simulink model "ferrucci299571_assign1_complete"  (R2026a)
settings: Solver=ode14x  StopTime=simTime  FixedStep=fixedStepSize
undefined symbols (not defined in the file or in its folder): RW
libraries: fl_lib x36, nesl_utility x12, ee_lib x3
settings Model: Creator=ferru  LastModifiedBy=ferru

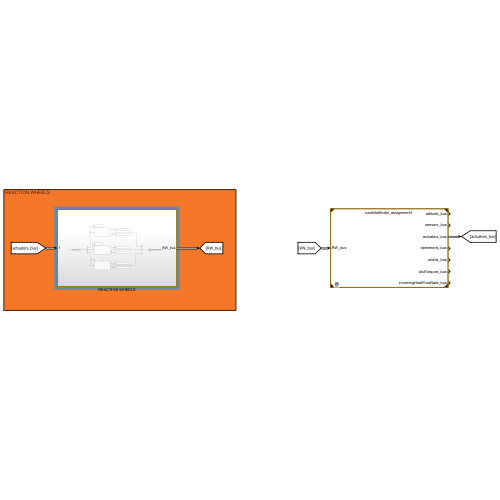
[thumbnail: Simulink's stored preview of the top-level diagram]
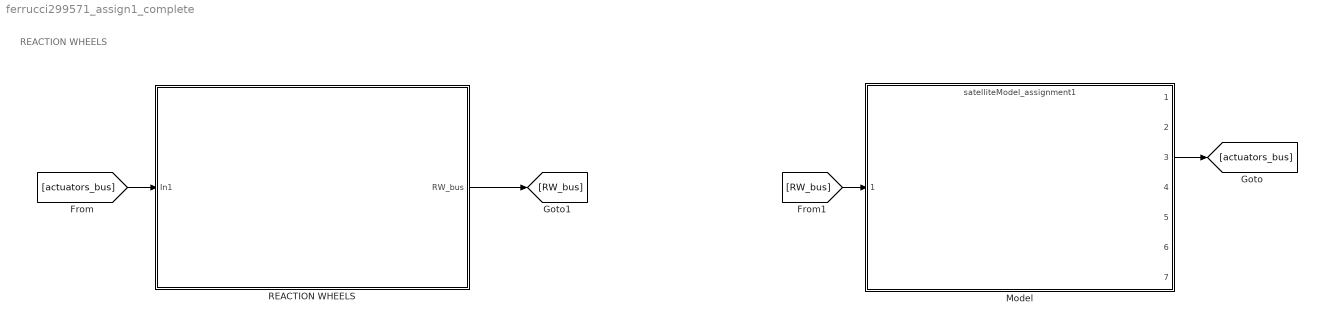
== system ferrucci299571_assign1_complete ==
  note: REACTION WHEELS
  Model : ModelReference  ModelNameDialog=satelliteModel_assignment1.slxp  ModelReferenceVersion=4.59  CopyOfModelProtected=on
  REACTION WHEELS : Subsystem
  wires:
  Model/3 -> [actuators_bus]
  [RW_bus] -> Model/1
  [actuators_bus] -> REACTION WHEELS/1(In1)
  REACTION WHEELS/1(RW_bus) -> [RW_bus]

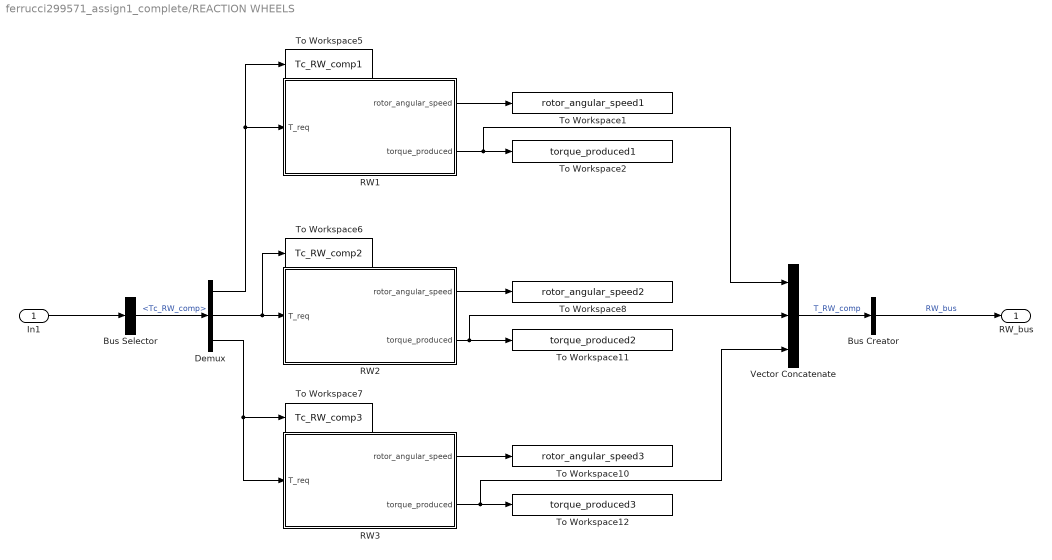
== system ferrucci299571_assign1_complete/REACTION WHEELS ==
  In1 : Inport
  Bus Creator : BusCreator  Inputs=1
  Bus Selector : BusSelector  OutputSignals=RW_bus.Tc_RW_comp
  Demux : Demux  Outputs=3
  RW1 : Subsystem
  RW2 : Subsystem
  RW3 : Subsystem
  To Workspace1 : ToWorkspace  VariableName=rotor_angular_speed1  SampleTime=-1
      settings: Save2DSignal=2-D array (concatenate along first dimension)
  To Workspace10 : ToWorkspace  VariableName=rotor_angular_speed3  SampleTime=-1
      settings: Save2DSignal=2-D array (concatenate along first dimension)
  To Workspace11 : ToWorkspace  VariableName=torque_produced2  SampleTime=-1
      settings: Save2DSignal=2-D array (concatenate along first dimension)
  To Workspace12 : ToWorkspace  VariableName=torque_produced3  SampleTime=-1
      settings: Save2DSignal=2-D array (concatenate along first dimension)
  To Workspace2 : ToWorkspace  VariableName=torque_produced1  SampleTime=-1
      settings: Save2DSignal=2-D array (concatenate along first dimension)
  To Workspace5 : ToWorkspace  VariableName=Tc_RW_comp1  SampleTime=-1
      settings: Save2DSignal=2-D array (concatenate along first dimension)
  To Workspace6 : ToWorkspace  VariableName=Tc_RW_comp2  SampleTime=-1
      settings: Save2DSignal=2-D array (concatenate along first dimension)
  To Workspace7 : ToWorkspace  VariableName=Tc_RW_comp3  SampleTime=-1
      settings: Save2DSignal=2-D array (concatenate along first dimension)
  To Workspace8 : ToWorkspace  VariableName=rotor_angular_speed2  SampleTime=-1
      settings: Save2DSignal=2-D array (concatenate along first dimension)
  Vector Concatenate : Concatenate  NumInputs=3  Mode=Multidimensional array
  RW_bus : Outport
  wires:
  Vector Concatenate/1 -> Bus Creator/1  "T_RW_comp"
  Demux/1 -> To Workspace5/1, RW1/1(T_req)
  Demux/3 -> RW3/1(T_req), To Workspace7/1
  Bus Creator/1 -> RW_bus/1  "RW_bus"
  RW3/2(torque_produced) -> Vector Concatenate/3, To Workspace12/1
  Bus Selector/1 -> Demux/1  "<Tc_RW_comp>"
  RW1/1(rotor_angular_speed) -> To Workspace1/1
  RW3/1(rotor_angular_speed) -> To Workspace10/1
  Demux/2 -> RW2/1(T_req), To Workspace6/1
  RW2/2(torque_produced) -> Vector Concatenate/2, To Workspace11/1
  RW2/1(rotor_angular_speed) -> To Workspace8/1
  RW1/2(torque_produced) -> Vector Concatenate/1, To Workspace2/1
  In1/1 -> Bus Selector/1

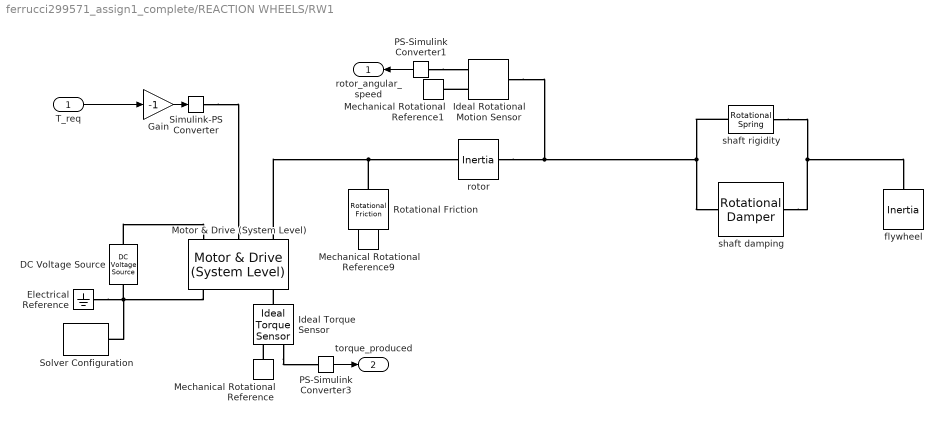
== system ferrucci299571_assign1_complete/REACTION WHEELS/RW1 ==
  T_req : Inport
  DC Voltage Source : fl_lib/Electrical/Electrical Sources/DC Voltage Source  v0=10 V
  Electrical Reference : fl_lib/Electrical/Electrical Elements/Electrical Reference
  Gain : Gain  Gain=-1
  Ideal Rotational Motion Sensor : fl_lib/Mechanical/Mechanical Sensors/Ideal Rotational Motion Sensor  reference=foundation.enum.MeasurementReference.difference  acceleration_port=false  velocity_port=true  position_port=false  wrap_angle=false  offset=0 rad
  Ideal Torque Sensor : fl_lib/Mechanical/Mechanical Sensors/Ideal Torque Sensor
  Mechanical Rotational Reference : fl_lib/Mechanical/Rotational Elements/Mechanical Rotational Reference
  Mechanical Rotational Reference1 : fl_lib/Mechanical/Rotational Elements/Mechanical Rotational Reference
  Mechanical Rotational Reference9 : fl_lib/Mechanical/Rotational Elements/Mechanical Rotational Reference
  Motor & Drive (System Level) : ee_lib/Electromechanical/Motor & Drive (System Level)  torque_speed_param=ee.enum.electromech.envelope.tabulated  overtorque_param=ee.enum.electromech.overtorque.no  T_t=RW.torque_envelope_val mN*m  T_t_intermittent=[.36, .32, .28, 0] N*m  T_t_2D=[.09, .09, .09; .08, .08, .08; .07, .07, .07; 0, 0, 0] N*m  T_t_intermittent_2D=[.36, .36, .36; .32, .32, .32; .28, .28, .28; 0, 0, 0] N*m  w_t=RW.torque_envelope_omega rad/s  vdc_t=[6, 12, 24] V  torque_max=0.1 N*m  power_max=30 W  torque_max_intermittent=0.4 N*m  power_max_intermittent=120 W  time_overtorque=30 s  time_recover=60 s  Tc=RW.torque_control_tc s  EnableSwitch=false  losses_param=ee.enum.electromech.motorAndDrive.lossParameterization.TabulatedEfficiencyDataAsAFunctionOfSpeedAndTorque  eff=100  w_eff=3750 rpm  T_eff=0.08 N*m  Piron=0 W  Pbase=0 W  w_eff_vec=RW.efficiency_omega rad/s  T_eff_vec=RW.efficiency_torque mN*m  v_eff_vec=[100, 250, 400] V  losses_mat=[1.49, 1.67, 2.21, 3.1; .42, .69, 1.14, 2.03; .06, .24, .78, 1.68; .42, .69, 1.14, 2.03; 1.49, 1.67, 2.21, 3.1] W  efficiency_mat=RW.efficiency_mat  losses_mat_3D=ones(5, 4, 3) W  efficiency_mat_3D=95 * ones(5, 4, 3)  Res=0 Ohm  J=RW.rotor_inertia_motor kg*m^2  lam=RW.rotor_damping N*m*s/rad  speed0=0 rpm  faulted_specify=off  faulted_priority=None  faulted=0  faulted_nominal_specify=off  faulted_nominal_value=1  faulted_nominal_unit=1  isSwitchedOff_specify=off  isSwitchedOff_priority=None  isSwitchedOff=0  isSwitchedOff_nominal_specify=off  isSwitchedOff_nominal_value=1  isSwitchedOff_nominal_unit=1  torqueLimitContinuous_specify=off  torqueLimitContinuous_priority=None  torqueLimitContinuous=0 N*m  torqueLimitContinuous_nominal_specify=off  torqueLimitContinuous_nominal_value=1  torqueLimitContinuous_nominal_unit=N*m  TabulateLossesForMultipleTemperatures=false  alpha=3.93e-3 1/K  Tmeas=25 degC  TmeasVec=[25, 75, 125] degC  Tmeas2=125 degC  losses_mat_T2=[1.49, 1.74, 2.49, 3.74; .42, .67, 1.42, 2.67; .06, .31, 1.06, 2.31; .42, .67, 1.42, 2.67; 1.49, 1.74, 2.49, 3.74] W  efficiency_mat_T2=[95, 95, 95, 95; 95, 95, 95, 95; 95, 95, 95, 95; 95, 95, 95, 95; 95, 95, 95, 95]  losses_mat_3D_T2=ones(5, 4, 3) W  efficiency_mat_3D_T2=95 * ones(5, 4, 3)  lossesMatMultipleTemperatures=ones(5, 4, 3) W  efficiencyMatMultipleTemperatures=95 * ones(5, 4, 3)  lossesMat4DMultipleTemperatures=ones(5, 4, 3, 3) W  efficiencyMat4DMultipleTemperatures=95 * ones(5, 4, 3, 3)  thermal_mass=100 J/K  initial_temperature=25 degC
  PS-Simulink Converter1 : nesl_utility/PS-Simulink Converter  PhysicalDomain=network_engine_domain  SubClassName=ps_output  LeftPortType=input  RightPortType=output  PseudoPeriodic=off  Frequencies=[]  VectorFormat=inherit  Unit=rad/s  AffineConversion=off
  PS-Simulink Converter3 : nesl_utility/PS-Simulink Converter  PhysicalDomain=network_engine_domain  SubClassName=ps_output  LeftPortType=input  RightPortType=output  PseudoPeriodic=off  Frequencies=[]  VectorFormat=inherit  Unit=N*m  AffineConversion=off
  Rotational Friction : fl_lib/Mechanical/Rotational Elements/Rotational Friction  brkwy_trq=RW.breakaway_friction_torque N*m  brkwy_vel=RW.breakaway_friction_velocity rad/s  Col_trq=RW.coulomb_friction_torque N*m  visc_coef=RW.viscous_friction_coeff N*m*s/rad  w_specify=off  w_priority=None  w=0 rad/s  w_nominal_specify=off  w_nominal_value=1  w_nominal_unit=rad/s  t_specify=off  t_priority=None  t=0 N*m  t_nominal_specify=off  t_nominal_value=1  t_nominal_unit=N*m
  Simulink-PS Converter : nesl_utility/Simulink-PS Converter  PhysicalDomain=network_engine_domain  SubClassName=ps_input  LeftPortType=input  RightPortType=output  PseudoPeriodic=off  Frequencies=[]  NoiseDistribution=none  NoiseParameters=[]  Unit=N*m  AffineConversion=off  FilteringAndDerivatives=provide  SimscapeFilterOrder=1  InputFilterTimeConstant=0.001  UdotUserProvided=0
  Solver Configuration : nesl_utility/Solver Configuration  PhysicalDomain=network_engine_domain  SubClassName=solver  LeftPortType=input  RightPortType=generic  Tones=[]  Harmonics=[]  SimulateNoise=off  Profile=off  UseLocalSampling=off  EnableSwitchedLinearOptims=on  FrequencyDomain=off  UseCCode=off  RelTol=0.001  AbsTol=0.001  MinStep=1e-09  ToWorkspace=off  RevertToSquareIcSolve=off  NumHomotopyIterations=100  PhasorMode=off  PhasorModeNumHarmonics=1  ConsistencySolver=NEWTON_XTOL_AFTER_FTOL  CanonicalOrdering=CANONICAL  OptimizeIntermediates=OPTIMIZED  IndexReductionMethod=DerivativeReplacement  DoDC=off  ResidualTolerance=1e-09  ConsistencyTolSource=GLOBAL  ConsistencyAbsTol=0.001  ConsistencyRelTol=0.001  ConsistencyTolFactor=0.001  UseLocalSolver=off  LocalSolverChoice=NE_BACKWARD_EULER_ADVANCER  ResolveIndetEquations=on  FunctionEvalNumThread=1  LocalSolverSampleTime=0.001  DoFixedCost=off  MaxNonlinIter=3  MaxModeIter=2  ComputeImpulses=off  ImpulseIterations=2  LinearAlgebra=auto  LinearAlgebraNumThread=0  EquationFormulation=NE_TIME_EF  DelaysMemoryBudget=1024  AutomaticFiltering=on  FilteringTimeConstant=0.001  PartitionStorageMethod=AS_NEEDED  PartitionMemoryBudget=1024  PartitionMethod=ROBUST  MultibodyUseLocalSolver=off  MultibodyLocalSolverChoice=ODE1  MultibodyLocalSolverSampleTime=0.001
  flywheel : fl_lib/Mechanical/Rotational Elements/Inertia  inertia=RW.flywheel_inertia kg*m^2  num_ports=foundation.enum.numPorts2.one  w_specify=off  w_priority=High  w=0 rad/s  w_nominal_specify=off  w_nominal_value=1  w_nominal_unit=rad/s  t_specify=off  t_priority=None  t=0 N*m  t_nominal_specify=off  t_nominal_value=1  t_nominal_unit=N*m
  rotor : fl_lib/Mechanical/Rotational Elements/Inertia  inertia=RW.rotor_inertia kg*m^2  num_ports=foundation.enum.numPorts2.two  w_specify=off  w_priority=High  w=0 rad/s  w_nominal_specify=off  w_nominal_value=1  w_nominal_unit=rad/s  t_specify=off  t_priority=None  t=0 N*m  t_nominal_specify=off  t_nominal_value=1  t_nominal_unit=N*m
  shaft damping : fl_lib/Mechanical/Rotational Elements/Rotational Damper  D=RW.shaft_damping_coeff N*m*s/rad  w_specify=off  w_priority=None  w=0 rad/s  w_nominal_specify=off  w_nominal_value=1  w_nominal_unit=rad/s  t_specify=off  t_priority=None  t=0 N*m  t_nominal_specify=off  t_nominal_value=1  t_nominal_unit=N*m
  shaft rigidity : fl_lib/Mechanical/Rotational Elements/Rotational Spring  spr_rate=RW.shaft_spring_rate N*m/rad  w_specify=off  w_priority=None  w=0 rad/s  w_nominal_specify=off  w_nominal_value=1  w_nominal_unit=rad/s  t_specify=off  t_priority=None  t=0 N*m  t_nominal_specify=off  t_nominal_value=1  t_nominal_unit=N*m  phi_specify=off  phi_priority=High  phi=0 rad  phi_nominal_specify=off  phi_nominal_value=1  phi_nominal_unit=rad
  rotor_angular_speed : Outport
  torque_produced : Outport  Port=2
  wires:
  Gain/1 -> Simulink-PS Converter/1
  PS-Simulink Converter3/1 -> torque_produced/1
  PS-Simulink Converter1/1 -> rotor_angular_speed/1
  T_req/1 -> Gain/1
  connections:
  DC Voltage Source/RConn1 -- Electrical Reference/LConn1 -- Motor & Drive (System Level)/RConn1 -- Solver Configuration/RConn1
  Mechanical Rotational Reference9/LConn1 -- Rotational Friction/RConn1
  Ideal Torque Sensor/RConn2 -- PS-Simulink Converter3/LConn1
  shaft rigidity/LConn1 -- flywheel/LConn1 -- shaft damping/LConn1
  Rotational Friction/LConn1 -- Motor & Drive (System Level)/LConn3 -- rotor/RConn1
  Simulink-PS Converter/RConn1 -- Motor & Drive (System Level)/LConn2
  PS-Simulink Converter1/LConn1 -- Ideal Rotational Motion Sensor/RConn2
  Mechanical Rotational Reference/LConn1 -- Ideal Torque Sensor/RConn1
  Ideal Rotational Motion Sensor/RConn1 -- Mechanical Rotational Reference1/LConn1
  DC Voltage Source/LConn1 -- Motor & Drive (System Level)/LConn1
  rotor/LConn1 -- Ideal Rotational Motion Sensor/LConn1 -- shaft rigidity/RConn1 -- shaft damping/RConn1
  Ideal Torque Sensor/LConn1 -- Motor & Drive (System Level)/RConn3

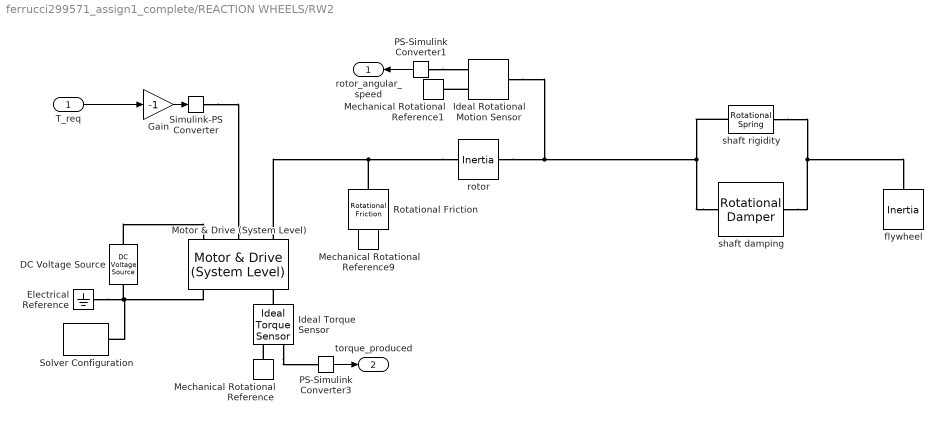
== system ferrucci299571_assign1_complete/REACTION WHEELS/RW2 ==
  T_req : Inport
  DC Voltage Source : fl_lib/Electrical/Electrical Sources/DC Voltage Source  v0=10 V
  Electrical Reference : fl_lib/Electrical/Electrical Elements/Electrical Reference
  Gain : Gain  Gain=-1
  Ideal Rotational Motion Sensor : fl_lib/Mechanical/Mechanical Sensors/Ideal Rotational Motion Sensor  reference=foundation.enum.MeasurementReference.difference  acceleration_port=false  velocity_port=true  position_port=false  wrap_angle=false  offset=0 rad
  Ideal Torque Sensor : fl_lib/Mechanical/Mechanical Sensors/Ideal Torque Sensor
  Mechanical Rotational Reference : fl_lib/Mechanical/Rotational Elements/Mechanical Rotational Reference
  Mechanical Rotational Reference1 : fl_lib/Mechanical/Rotational Elements/Mechanical Rotational Reference
  Mechanical Rotational Reference9 : fl_lib/Mechanical/Rotational Elements/Mechanical Rotational Reference
  Motor & Drive (System Level) : ee_lib/Electromechanical/Motor & Drive (System Level)  torque_speed_param=ee.enum.electromech.envelope.tabulated  overtorque_param=ee.enum.electromech.overtorque.no  T_t=RW.torque_envelope_val mN*m  T_t_intermittent=[.36, .32, .28, 0] N*m  T_t_2D=[.09, .09, .09; .08, .08, .08; .07, .07, .07; 0, 0, 0] N*m  T_t_intermittent_2D=[.36, .36, .36; .32, .32, .32; .28, .28, .28; 0, 0, 0] N*m  w_t=RW.torque_envelope_omega rad/s  vdc_t=[6, 12, 24] V  torque_max=0.1 N*m  power_max=30 W  torque_max_intermittent=0.4 N*m  power_max_intermittent=120 W  time_overtorque=30 s  time_recover=60 s  Tc=RW.torque_control_tc s  EnableSwitch=false  losses_param=ee.enum.electromech.motorAndDrive.lossParameterization.TabulatedEfficiencyDataAsAFunctionOfSpeedAndTorque  eff=100  w_eff=3750 rpm  T_eff=0.08 N*m  Piron=0 W  Pbase=0 W  w_eff_vec=RW.efficiency_omega rad/s  T_eff_vec=RW.efficiency_torque mN*m  v_eff_vec=[100, 250, 400] V  losses_mat=[1.49, 1.67, 2.21, 3.1; .42, .69, 1.14, 2.03; .06, .24, .78, 1.68; .42, .69, 1.14, 2.03; 1.49, 1.67, 2.21, 3.1] W  efficiency_mat=RW.efficiency_mat  losses_mat_3D=ones(5, 4, 3) W  efficiency_mat_3D=95 * ones(5, 4, 3)  Res=0 Ohm  J=RW.rotor_inertia_motor kg*m^2  lam=RW.rotor_damping N*m*s/rad  speed0=0 rpm  faulted_specify=off  faulted_priority=None  faulted=0  faulted_nominal_specify=off  faulted_nominal_value=1  faulted_nominal_unit=1  isSwitchedOff_specify=off  isSwitchedOff_priority=None  isSwitchedOff=0  isSwitchedOff_nominal_specify=off  isSwitchedOff_nominal_value=1  isSwitchedOff_nominal_unit=1  torqueLimitContinuous_specify=off  torqueLimitContinuous_priority=None  torqueLimitContinuous=0 N*m  torqueLimitContinuous_nominal_specify=off  torqueLimitContinuous_nominal_value=1  torqueLimitContinuous_nominal_unit=N*m  TabulateLossesForMultipleTemperatures=false  alpha=3.93e-3 1/K  Tmeas=25 degC  TmeasVec=[25, 75, 125] degC  Tmeas2=125 degC  losses_mat_T2=[1.49, 1.74, 2.49, 3.74; .42, .67, 1.42, 2.67; .06, .31, 1.06, 2.31; .42, .67, 1.42, 2.67; 1.49, 1.74, 2.49, 3.74] W  efficiency_mat_T2=[95, 95, 95, 95; 95, 95, 95, 95; 95, 95, 95, 95; 95, 95, 95, 95; 95, 95, 95, 95]  losses_mat_3D_T2=ones(5, 4, 3) W  efficiency_mat_3D_T2=95 * ones(5, 4, 3)  lossesMatMultipleTemperatures=ones(5, 4, 3) W  efficiencyMatMultipleTemperatures=95 * ones(5, 4, 3)  lossesMat4DMultipleTemperatures=ones(5, 4, 3, 3) W  efficiencyMat4DMultipleTemperatures=95 * ones(5, 4, 3, 3)  thermal_mass=100 J/K  initial_temperature=25 degC
  PS-Simulink Converter1 : nesl_utility/PS-Simulink Converter  PhysicalDomain=network_engine_domain  SubClassName=ps_output  LeftPortType=input  RightPortType=output  PseudoPeriodic=off  Frequencies=[]  VectorFormat=inherit  Unit=rad/s  AffineConversion=off
  PS-Simulink Converter3 : nesl_utility/PS-Simulink Converter  PhysicalDomain=network_engine_domain  SubClassName=ps_output  LeftPortType=input  RightPortType=output  PseudoPeriodic=off  Frequencies=[]  VectorFormat=inherit  Unit=N*m  AffineConversion=off
  Rotational Friction : fl_lib/Mechanical/Rotational Elements/Rotational Friction  brkwy_trq=RW.breakaway_friction_torque N*m  brkwy_vel=RW.breakaway_friction_velocity rad/s  Col_trq=RW.coulomb_friction_torque N*m  visc_coef=RW.viscous_friction_coeff N*m*s/rad  w_specify=off  w_priority=None  w=0 rad/s  w_nominal_specify=off  w_nominal_value=1  w_nominal_unit=rad/s  t_specify=off  t_priority=None  t=0 N*m  t_nominal_specify=off  t_nominal_value=1  t_nominal_unit=N*m
  Simulink-PS Converter : nesl_utility/Simulink-PS Converter  PhysicalDomain=network_engine_domain  SubClassName=ps_input  LeftPortType=input  RightPortType=output  PseudoPeriodic=off  Frequencies=[]  NoiseDistribution=none  NoiseParameters=[]  Unit=N*m  AffineConversion=off  FilteringAndDerivatives=provide  SimscapeFilterOrder=1  InputFilterTimeConstant=0.001  UdotUserProvided=0
  Solver Configuration : nesl_utility/Solver Configuration  PhysicalDomain=network_engine_domain  SubClassName=solver  LeftPortType=input  RightPortType=generic  Tones=[]  Harmonics=[]  SimulateNoise=off  Profile=off  UseLocalSampling=off  EnableSwitchedLinearOptims=on  FrequencyDomain=off  UseCCode=off  RelTol=0.001  AbsTol=0.001  MinStep=1e-09  ToWorkspace=off  RevertToSquareIcSolve=off  NumHomotopyIterations=100  PhasorMode=off  PhasorModeNumHarmonics=1  ConsistencySolver=NEWTON_XTOL_AFTER_FTOL  CanonicalOrdering=CANONICAL  OptimizeIntermediates=OPTIMIZED  IndexReductionMethod=DerivativeReplacement  DoDC=off  ResidualTolerance=1e-09  ConsistencyTolSource=GLOBAL  ConsistencyAbsTol=0.001  ConsistencyRelTol=0.001  ConsistencyTolFactor=0.001  UseLocalSolver=off  LocalSolverChoice=NE_BACKWARD_EULER_ADVANCER  ResolveIndetEquations=on  FunctionEvalNumThread=1  LocalSolverSampleTime=0.001  DoFixedCost=off  MaxNonlinIter=3  MaxModeIter=2  ComputeImpulses=off  ImpulseIterations=2  LinearAlgebra=auto  LinearAlgebraNumThread=0  EquationFormulation=NE_TIME_EF  DelaysMemoryBudget=1024  AutomaticFiltering=on  FilteringTimeConstant=0.001  PartitionStorageMethod=AS_NEEDED  PartitionMemoryBudget=1024  PartitionMethod=ROBUST  MultibodyUseLocalSolver=off  MultibodyLocalSolverChoice=ODE1  MultibodyLocalSolverSampleTime=0.001
  flywheel : fl_lib/Mechanical/Rotational Elements/Inertia  inertia=RW.flywheel_inertia kg*m^2  num_ports=foundation.enum.numPorts2.one  w_specify=off  w_priority=High  w=0 rad/s  w_nominal_specify=off  w_nominal_value=1  w_nominal_unit=rad/s  t_specify=off  t_priority=None  t=0 N*m  t_nominal_specify=off  t_nominal_value=1  t_nominal_unit=N*m
  rotor : fl_lib/Mechanical/Rotational Elements/Inertia  inertia=RW.rotor_inertia kg*m^2  num_ports=foundation.enum.numPorts2.two  w_specify=off  w_priority=High  w=0 rad/s  w_nominal_specify=off  w_nominal_value=1  w_nominal_unit=rad/s  t_specify=off  t_priority=None  t=0 N*m  t_nominal_specify=off  t_nominal_value=1  t_nominal_unit=N*m
  shaft damping : fl_lib/Mechanical/Rotational Elements/Rotational Damper  D=RW.shaft_damping_coeff N*m*s/rad  w_specify=off  w_priority=None  w=0 rad/s  w_nominal_specify=off  w_nominal_value=1  w_nominal_unit=rad/s  t_specify=off  t_priority=None  t=0 N*m  t_nominal_specify=off  t_nominal_value=1  t_nominal_unit=N*m
  shaft rigidity : fl_lib/Mechanical/Rotational Elements/Rotational Spring  spr_rate=RW.shaft_spring_rate N*m/rad  w_specify=off  w_priority=None  w=0 rad/s  w_nominal_specify=off  w_nominal_value=1  w_nominal_unit=rad/s  t_specify=off  t_priority=None  t=0 N*m  t_nominal_specify=off  t_nominal_value=1  t_nominal_unit=N*m  phi_specify=off  phi_priority=High  phi=0 rad  phi_nominal_specify=off  phi_nominal_value=1  phi_nominal_unit=rad
  rotor_angular_speed : Outport
  torque_produced : Outport  Port=2
  wires:
  T_req/1 -> Gain/1
  PS-Simulink Converter1/1 -> rotor_angular_speed/1
  PS-Simulink Converter3/1 -> torque_produced/1
  Gain/1 -> Simulink-PS Converter/1
  connections:
  Ideal Torque Sensor/LConn1 -- Motor & Drive (System Level)/RConn3
  shaft damping/RConn1 -- shaft rigidity/RConn1 -- Ideal Rotational Motion Sensor/LConn1 -- rotor/LConn1
  DC Voltage Source/LConn1 -- Motor & Drive (System Level)/LConn1
  Ideal Rotational Motion Sensor/RConn1 -- Mechanical Rotational Reference1/LConn1
  Mechanical Rotational Reference/LConn1 -- Ideal Torque Sensor/RConn1
  PS-Simulink Converter1/LConn1 -- Ideal Rotational Motion Sensor/RConn2
  Simulink-PS Converter/RConn1 -- Motor & Drive (System Level)/LConn2
  rotor/RConn1 -- Motor & Drive (System Level)/LConn3 -- Rotational Friction/LConn1
  shaft damping/LConn1 -- flywheel/LConn1 -- shaft rigidity/LConn1
  Ideal Torque Sensor/RConn2 -- PS-Simulink Converter3/LConn1
  Mechanical Rotational Reference9/LConn1 -- Rotational Friction/RConn1
  Solver Configuration/RConn1 -- Motor & Drive (System Level)/RConn1 -- Electrical Reference/LConn1 -- DC Voltage Source/RConn1

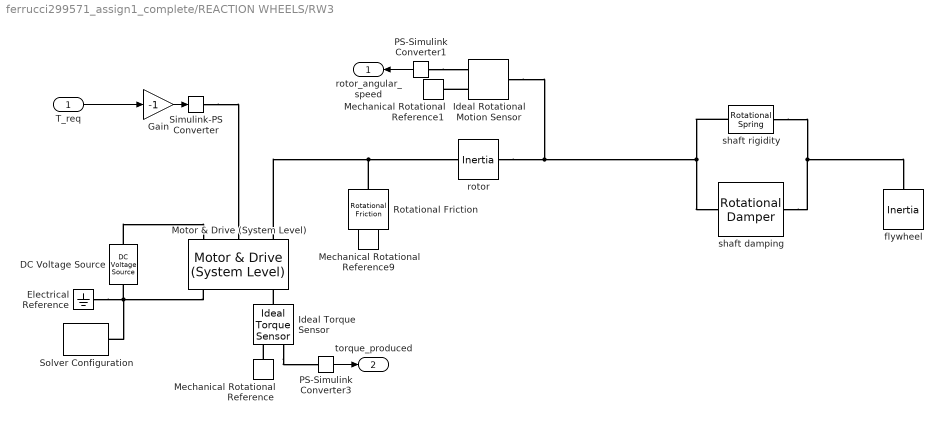
== system ferrucci299571_assign1_complete/REACTION WHEELS/RW3 ==
  T_req : Inport
  DC Voltage Source : fl_lib/Electrical/Electrical Sources/DC Voltage Source  v0=10 V
  Electrical Reference : fl_lib/Electrical/Electrical Elements/Electrical Reference
  Gain : Gain  Gain=-1
  Ideal Rotational Motion Sensor : fl_lib/Mechanical/Mechanical Sensors/Ideal Rotational Motion Sensor  reference=foundation.enum.MeasurementReference.difference  acceleration_port=false  velocity_port=true  position_port=false  wrap_angle=false  offset=0 rad
  Ideal Torque Sensor : fl_lib/Mechanical/Mechanical Sensors/Ideal Torque Sensor
  Mechanical Rotational Reference : fl_lib/Mechanical/Rotational Elements/Mechanical Rotational Reference
  Mechanical Rotational Reference1 : fl_lib/Mechanical/Rotational Elements/Mechanical Rotational Reference
  Mechanical Rotational Reference9 : fl_lib/Mechanical/Rotational Elements/Mechanical Rotational Reference
  Motor & Drive (System Level) : ee_lib/Electromechanical/Motor & Drive (System Level)  torque_speed_param=ee.enum.electromech.envelope.tabulated  overtorque_param=ee.enum.electromech.overtorque.no  T_t=RW.torque_envelope_val mN*m  T_t_intermittent=[.36, .32, .28, 0] N*m  T_t_2D=[.09, .09, .09; .08, .08, .08; .07, .07, .07; 0, 0, 0] N*m  T_t_intermittent_2D=[.36, .36, .36; .32, .32, .32; .28, .28, .28; 0, 0, 0] N*m  w_t=RW.torque_envelope_omega rad/s  vdc_t=[6, 12, 24] V  torque_max=0.1 N*m  power_max=30 W  torque_max_intermittent=0.4 N*m  power_max_intermittent=120 W  time_overtorque=30 s  time_recover=60 s  Tc=RW.torque_control_tc s  EnableSwitch=false  losses_param=ee.enum.electromech.motorAndDrive.lossParameterization.TabulatedEfficiencyDataAsAFunctionOfSpeedAndTorque  eff=100  w_eff=3750 rpm  T_eff=0.08 N*m  Piron=0 W  Pbase=0 W  w_eff_vec=RW.efficiency_omega rad/s  T_eff_vec=RW.efficiency_torque mN*m  v_eff_vec=[100, 250, 400] V  losses_mat=[1.49, 1.67, 2.21, 3.1; .42, .69, 1.14, 2.03; .06, .24, .78, 1.68; .42, .69, 1.14, 2.03; 1.49, 1.67, 2.21, 3.1] W  efficiency_mat=RW.efficiency_mat  losses_mat_3D=ones(5, 4, 3) W  efficiency_mat_3D=95 * ones(5, 4, 3)  Res=0 Ohm  J=RW.rotor_inertia_motor kg*m^2  lam=RW.rotor_damping N*m*s/rad  speed0=0 rpm  faulted_specify=off  faulted_priority=None  faulted=0  faulted_nominal_specify=off  faulted_nominal_value=1  faulted_nominal_unit=1  isSwitchedOff_specify=off  isSwitchedOff_priority=None  isSwitchedOff=0  isSwitchedOff_nominal_specify=off  isSwitchedOff_nominal_value=1  isSwitchedOff_nominal_unit=1  torqueLimitContinuous_specify=off  torqueLimitContinuous_priority=None  torqueLimitContinuous=0 N*m  torqueLimitContinuous_nominal_specify=off  torqueLimitContinuous_nominal_value=1  torqueLimitContinuous_nominal_unit=N*m  TabulateLossesForMultipleTemperatures=false  alpha=3.93e-3 1/K  Tmeas=25 degC  TmeasVec=[25, 75, 125] degC  Tmeas2=125 degC  losses_mat_T2=[1.49, 1.74, 2.49, 3.74; .42, .67, 1.42, 2.67; .06, .31, 1.06, 2.31; .42, .67, 1.42, 2.67; 1.49, 1.74, 2.49, 3.74] W  efficiency_mat_T2=[95, 95, 95, 95; 95, 95, 95, 95; 95, 95, 95, 95; 95, 95, 95, 95; 95, 95, 95, 95]  losses_mat_3D_T2=ones(5, 4, 3) W  efficiency_mat_3D_T2=95 * ones(5, 4, 3)  lossesMatMultipleTemperatures=ones(5, 4, 3) W  efficiencyMatMultipleTemperatures=95 * ones(5, 4, 3)  lossesMat4DMultipleTemperatures=ones(5, 4, 3, 3) W  efficiencyMat4DMultipleTemperatures=95 * ones(5, 4, 3, 3)  thermal_mass=100 J/K  initial_temperature=25 degC
  PS-Simulink Converter1 : nesl_utility/PS-Simulink Converter  PhysicalDomain=network_engine_domain  SubClassName=ps_output  LeftPortType=input  RightPortType=output  PseudoPeriodic=off  Frequencies=[]  VectorFormat=inherit  Unit=rad/s  AffineConversion=off
  PS-Simulink Converter3 : nesl_utility/PS-Simulink Converter  PhysicalDomain=network_engine_domain  SubClassName=ps_output  LeftPortType=input  RightPortType=output  PseudoPeriodic=off  Frequencies=[]  VectorFormat=inherit  Unit=N*m  AffineConversion=off
  Rotational Friction : fl_lib/Mechanical/Rotational Elements/Rotational Friction  brkwy_trq=RW.breakaway_friction_torque N*m  brkwy_vel=RW.breakaway_friction_velocity rad/s  Col_trq=RW.coulomb_friction_torque N*m  visc_coef=RW.viscous_friction_coeff N*m*s/rad  w_specify=off  w_priority=None  w=0 rad/s  w_nominal_specify=off  w_nominal_value=1  w_nominal_unit=rad/s  t_specify=off  t_priority=None  t=0 N*m  t_nominal_specify=off  t_nominal_value=1  t_nominal_unit=N*m
  Simulink-PS Converter : nesl_utility/Simulink-PS Converter  PhysicalDomain=network_engine_domain  SubClassName=ps_input  LeftPortType=input  RightPortType=output  PseudoPeriodic=off  Frequencies=[]  NoiseDistribution=none  NoiseParameters=[]  Unit=N*m  AffineConversion=off  FilteringAndDerivatives=provide  SimscapeFilterOrder=1  InputFilterTimeConstant=0.001  UdotUserProvided=0
  Solver Configuration : nesl_utility/Solver Configuration  PhysicalDomain=network_engine_domain  SubClassName=solver  LeftPortType=input  RightPortType=generic  Tones=[]  Harmonics=[]  SimulateNoise=off  Profile=off  UseLocalSampling=off  EnableSwitchedLinearOptims=on  FrequencyDomain=off  UseCCode=off  RelTol=0.001  AbsTol=0.001  MinStep=1e-09  ToWorkspace=off  RevertToSquareIcSolve=off  NumHomotopyIterations=100  PhasorMode=off  PhasorModeNumHarmonics=1  ConsistencySolver=NEWTON_XTOL_AFTER_FTOL  CanonicalOrdering=CANONICAL  OptimizeIntermediates=OPTIMIZED  IndexReductionMethod=DerivativeReplacement  DoDC=off  ResidualTolerance=1e-09  ConsistencyTolSource=GLOBAL  ConsistencyAbsTol=0.001  ConsistencyRelTol=0.001  ConsistencyTolFactor=0.001  UseLocalSolver=off  LocalSolverChoice=NE_BACKWARD_EULER_ADVANCER  ResolveIndetEquations=on  FunctionEvalNumThread=1  LocalSolverSampleTime=0.001  DoFixedCost=off  MaxNonlinIter=3  MaxModeIter=2  ComputeImpulses=off  ImpulseIterations=2  LinearAlgebra=auto  LinearAlgebraNumThread=0  EquationFormulation=NE_TIME_EF  DelaysMemoryBudget=1024  AutomaticFiltering=on  FilteringTimeConstant=0.001  PartitionStorageMethod=AS_NEEDED  PartitionMemoryBudget=1024  PartitionMethod=ROBUST  MultibodyUseLocalSolver=off  MultibodyLocalSolverChoice=ODE1  MultibodyLocalSolverSampleTime=0.001
  flywheel : fl_lib/Mechanical/Rotational Elements/Inertia  inertia=RW.flywheel_inertia kg*m^2  num_ports=foundation.enum.numPorts2.one  w_specify=off  w_priority=High  w=0 rad/s  w_nominal_specify=off  w_nominal_value=1  w_nominal_unit=rad/s  t_specify=off  t_priority=None  t=0 N*m  t_nominal_specify=off  t_nominal_value=1  t_nominal_unit=N*m
  rotor : fl_lib/Mechanical/Rotational Elements/Inertia  inertia=RW.rotor_inertia kg*m^2  num_ports=foundation.enum.numPorts2.two  w_specify=off  w_priority=High  w=0 rad/s  w_nominal_specify=off  w_nominal_value=1  w_nominal_unit=rad/s  t_specify=off  t_priority=None  t=0 N*m  t_nominal_specify=off  t_nominal_value=1  t_nominal_unit=N*m
  shaft damping : fl_lib/Mechanical/Rotational Elements/Rotational Damper  D=RW.shaft_damping_coeff N*m*s/rad  w_specify=off  w_priority=None  w=0 rad/s  w_nominal_specify=off  w_nominal_value=1  w_nominal_unit=rad/s  t_specify=off  t_priority=None  t=0 N*m  t_nominal_specify=off  t_nominal_value=1  t_nominal_unit=N*m
  shaft rigidity : fl_lib/Mechanical/Rotational Elements/Rotational Spring  spr_rate=RW.shaft_spring_rate N*m/rad  w_specify=off  w_priority=None  w=0 rad/s  w_nominal_specify=off  w_nominal_value=1  w_nominal_unit=rad/s  t_specify=off  t_priority=None  t=0 N*m  t_nominal_specify=off  t_nominal_value=1  t_nominal_unit=N*m  phi_specify=off  phi_priority=High  phi=0 rad  phi_nominal_specify=off  phi_nominal_value=1  phi_nominal_unit=rad
  rotor_angular_speed : Outport
  torque_produced : Outport  Port=2
  wires:
  Gain/1 -> Simulink-PS Converter/1
  PS-Simulink Converter3/1 -> torque_produced/1
  PS-Simulink Converter1/1 -> rotor_angular_speed/1
  T_req/1 -> Gain/1
  connections:
  DC Voltage Source/RConn1 -- Electrical Reference/LConn1 -- Motor & Drive (System Level)/RConn1 -- Solver Configuration/RConn1
  Mechanical Rotational Reference9/LConn1 -- Rotational Friction/RConn1
  Ideal Torque Sensor/RConn2 -- PS-Simulink Converter3/LConn1
  shaft rigidity/LConn1 -- flywheel/LConn1 -- shaft damping/LConn1
  Rotational Friction/LConn1 -- Motor & Drive (System Level)/LConn3 -- rotor/RConn1
  Simulink-PS Converter/RConn1 -- Motor & Drive (System Level)/LConn2
  PS-Simulink Converter1/LConn1 -- Ideal Rotational Motion Sensor/RConn2
  Mechanical Rotational Reference/LConn1 -- Ideal Torque Sensor/RConn1
  Ideal Rotational Motion Sensor/RConn1 -- Mechanical Rotational Reference1/LConn1
  DC Voltage Source/LConn1 -- Motor & Drive (System Level)/LConn1
  rotor/LConn1 -- Ideal Rotational Motion Sensor/LConn1 -- shaft rigidity/RConn1 -- shaft damping/RConn1
  Ideal Torque Sensor/LConn1 -- Motor & Drive (System Level)/RConn3
